simulink model "simulink12"  (R2021b)
settings: Solver=VariableStepAuto  StartTime=0.0  StopTime=24.0  RelTol=1e-3
settings Model: Creator=13676840  LastModifiedBy=14571525

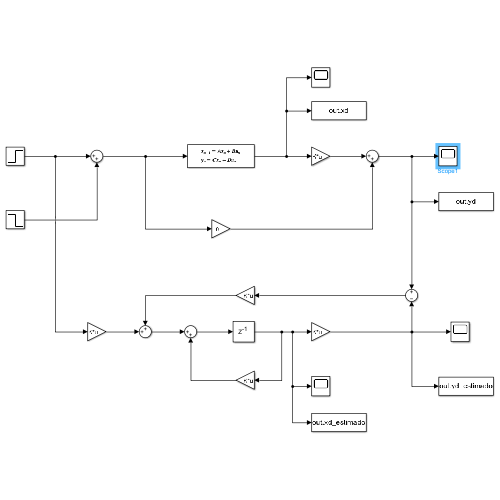
[thumbnail: Simulink's stored preview of the top-level diagram]
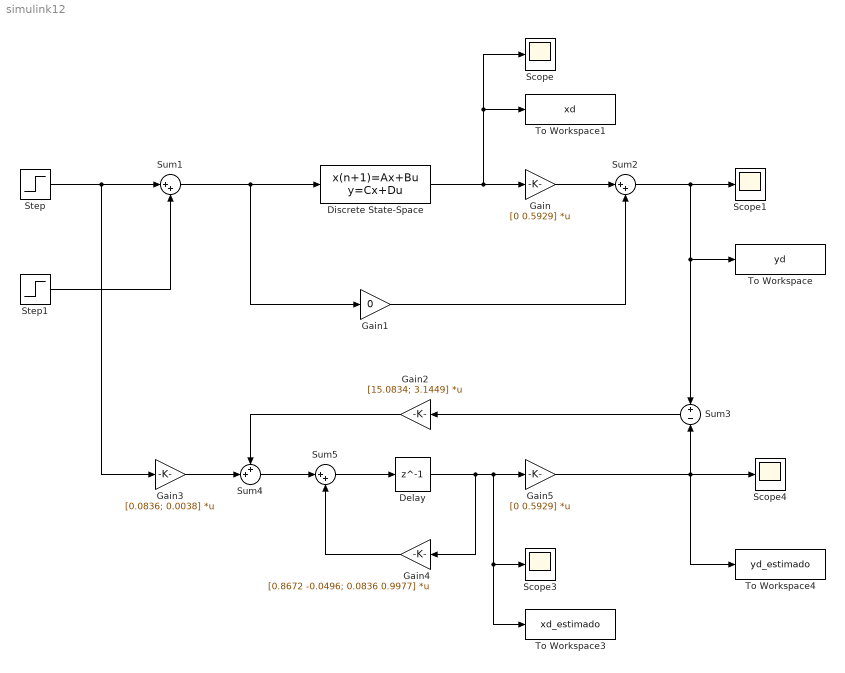
== system simulink12 ==
  Delay : Delay  DelayLength=1  InitialCondition=0
  Discrete State-Space : DiscreteStateSpace  A="[0.8672 -0.0496; 0.0836    0.9977]"  B=[0.0836; 0.0038]  C=[1 0; 0 1]  D=[0; 0]  InitialCondition=[-0.15 0.15]  SampleTime=0.2241
  Gain : Gain  Gain=[0 0.5929]  Multiplication=Matrix(K*u)
  Gain1 : Gain  Gain=0
  Gain2 : Gain  Gain=[15.0834; 3.1449]  Multiplication=Matrix(K*u)
  Gain3 : Gain  Gain=[0.0836; 0.0038]  Multiplication=Matrix(K*u)
  Gain4 : Gain  Gain=[0.8672 -0.0496; 0.0836 0.9977]  Multiplication=Matrix(K*u)
  Gain5 : Gain  Gain=[0 0.5929]  Multiplication=Matrix(K*u)
  Scope{,1,3..4} (4 alike) : Scope
  Step : Step  Time=0  After=1.17  SampleTime=0
  Step1 : Step  Time=12  After=-0.15  SampleTime=0
  Sum1 : Sum  Inputs=|++
  Sum2 : Sum  Inputs=|++
  Sum3 : Sum  Inputs=+|-
  Sum4 : Sum  Inputs=++|
  Sum5 : Sum  Inputs=|++
  To Workspace : ToWorkspace  VariableName=yd  SaveFormat=Timeseries  SampleTime=-1
  To Workspace1 : ToWorkspace  VariableName=xd  SaveFormat=Timeseries  SampleTime=-1
  To Workspace3 : ToWorkspace  VariableName=xd_estimado  SaveFormat=Timeseries  SampleTime=-1
  To Workspace4 : ToWorkspace  VariableName=yd_estimado  SaveFormat=Timeseries  SampleTime=-1
  wires:
  Step/1 -> Gain3/1, Sum1/1
  Step1/1 -> Sum1/2
  Discrete State-Space/1 -> Scope/1, To Workspace1/1, Gain/1
  Gain/1 -> Sum2/1
  Sum2/1 -> Sum3/1, To Workspace/1, Scope1/1
  Gain1/1 -> Sum2/2
  Sum1/1 -> Gain1/1, Discrete State-Space/1
  Sum3/1 -> Gain2/1
  Gain3/1 -> Sum4/2
  Gain2/1 -> Sum4/1
  Sum4/1 -> Sum5/1
  Sum5/1 -> Delay/1
  Gain4/1 -> Sum5/2
  Delay/1 -> Gain4/1, To Workspace3/1, Scope3/1, Gain5/1
  Gain5/1 -> Scope4/1, To Workspace4/1, Sum3/2
